simulink model "ClosedLoopSys"  (Simulink 8.4)
settings: Solver=ode1  StartTime=0.00  StopTime=60.00  FixedStep=T  RelTol=1e-5
values from neighbouring files (symbols this model uses):
  DAC_lim_l = 0    [heli.m]
  DAC_lim_u = 10    [heli.m]
  e_lim_l = -50*pi/180    (= -0.872664625997)    [heli.m]
  T = 0.015    [heli.m]
undefined symbols (not defined in the file or in its folder): Cr, kdfilt, Kdt, Kidt, U_e
settings Model: Creator=bjones  LastModifiedBy=bjones
settings DataIOCC: LimitDataPoints=off
settings OptimizationCC: BlockReduction=off  BooleanDataType=off
settings DebuggingCC: SaveWithParameterizedLinksMsg=none  SignalResolutionControl=TryResolveAllWithWarning  SolverPrmCheckMsg=none  MultiTaskDSMMsg=warning  MultiTaskCondExecSysMsg=none  StrictBusMsg=None
settings HardwareCC: TargetUnknown=on
settings RTWCC: IncludeERTFirstTime=on

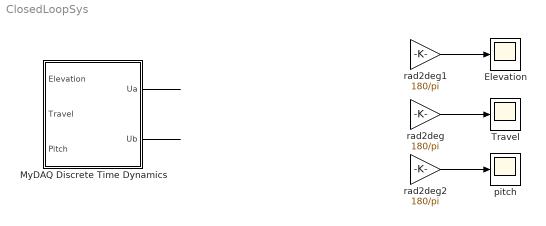
== system ClosedLoopSys ==
  Elevation : Scope
      settings: TimeRange=60  YMin=-50  YMax=30  SaveName=elev
  MyDAQ Discrete Time Dynamics : Subsystem
  Travel : Scope
      settings: TimeRange=60  YMin=-150  YMax=300  SaveName=trav
  pitch : Scope
      settings: TimeRange=60  YMin=-25  YMax=20  SaveName=pitch
  rad2deg : Gain  Gain=180/pi  SaturateOnIntegerOverflow=on  OutDataTypeStr=Inherit: Same as input  ParamDataTypeStr=Inherit: Same as input
  rad2deg1 : Gain  Gain=180/pi  SaturateOnIntegerOverflow=on  OutDataTypeStr=Inherit: Same as input  ParamDataTypeStr=Inherit: Same as input
  rad2deg2 : Gain  Gain=180/pi  SaturateOnIntegerOverflow=on  OutDataTypeStr=Inherit: Same as input  ParamDataTypeStr=Inherit: Same as input
  wires:
  rad2deg/1 -> Travel/1
  rad2deg1/1 -> Elevation/1
  ? -> MyDAQ Discrete Time Dynamics/2(Travel), rad2deg/1
  ? -> rad2deg1/1, MyDAQ Discrete Time Dynamics/1(Elevation)
  rad2deg2/1 -> pitch/1
  ? -> rad2deg2/1, MyDAQ Discrete Time Dynamics/3(Pitch)
  MyDAQ Discrete Time Dynamics/1(Ua) -> ?
  MyDAQ Discrete Time Dynamics/2(Ub) -> ?

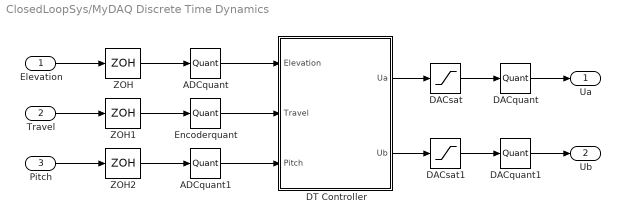
== system ClosedLoopSys/MyDAQ Discrete Time Dynamics ==
  Elevation : Inport
  Travel : Inport  Port=2
  Pitch : Inport  Port=3
  ADCquant : Quantizer  QuantizationInterval=ADC_Vres  SampleTime=T
  ADCquant1 : Quantizer  QuantizationInterval=ADC_Vres  SampleTime=T
  DACquant : Quantizer  QuantizationInterval=DAC_Vres  SampleTime=T
  DACquant1 : Quantizer  QuantizationInterval=DAC_Vres  SampleTime=T
  DACsat : Saturate  UpperLimit=DAC_lim_u  LowerLimit=DAC_lim_l  SampleTime=T
  DACsat1 : Saturate  UpperLimit=DAC_lim_u  LowerLimit=DAC_lim_l  SampleTime=T
  DT Controller : Subsystem
  Encoderquant : Quantizer  QuantizationInterval=Encoder_res  SampleTime=T
  ZOH : ZeroOrderHold  SampleTime=T
  ZOH1 : ZeroOrderHold  SampleTime=T
  ZOH2 : ZeroOrderHold  SampleTime=T
  Ua : Outport
  Ub : Outport  Port=2
  wires:
  Elevation/1 -> ZOH/1
  Travel/1 -> ZOH1/1
  DACquant/1 -> Ua/1
  DACquant1/1 -> Ub/1
  DT Controller/1(Ua) -> DACsat/1
  DACsat/1 -> DACquant/1
  DT Controller/2(Ub) -> DACsat1/1
  DACsat1/1 -> DACquant1/1
  ZOH1/1 -> Encoderquant/1
  ZOH/1 -> ADCquant/1
  Pitch/1 -> ZOH2/1
  ZOH2/1 -> ADCquant1/1
  ADCquant/1 -> DT Controller/1(Elevation)
  ADCquant1/1 -> DT Controller/3(Pitch)
  Encoderquant/1 -> DT Controller/2(Travel)

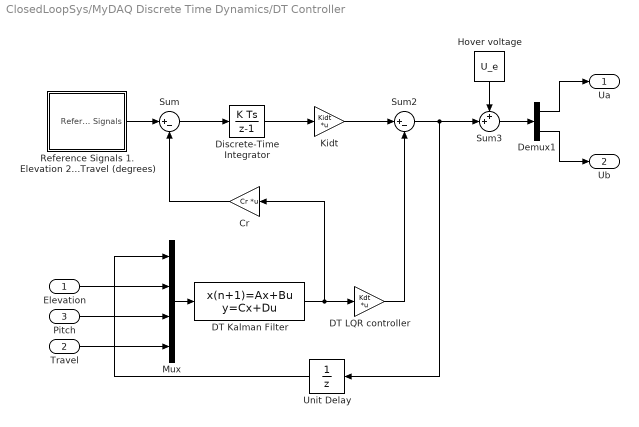
== system ClosedLoopSys/MyDAQ Discrete Time Dynamics/DT Controller ==
  Elevation : Inport
  Travel : Inport  Port=2
  Pitch : Inport  Port=3
  Cr : Gain  Gain=Cr  Multiplication=Matrix(K*u)
  DT Kalman Filter : DiscreteStateSpace  A=kdfilt.a  B=kdfilt.b  C=kdfilt.c(size(C,1)+1:end,:)  D=kdfilt.d(size(C,1)+1:end,:)  X0=[e_lim_l; 0; 0; 0; 0; 0]  SampleTime=T
  DT LQR controller : Gain  Gain=Kdt  Multiplication=Matrix(K*u)
  Demux1 : Demux  Outputs=2
  Discrete-Time Integrator : DiscreteIntegrator  SampleTime=T
  Hover voltage : Constant  Value=U_e  SampleTime=T
  Kidt : Gain  Gain=Kidt  Multiplication=Matrix(K*u)
  Mux : Mux
  Reference Signals 1. Elevation 2. Travel (degrees) : Subsystem
  Sum : Sum  Inputs=|+-  SampleTime=T
  Sum2 : Sum  Inputs=|+-  SampleTime=T
  Sum3 : Sum  Inputs=++|  SampleTime=T
  Unit Delay : UnitDelay  SampleTime=T
  Ua : Outport
  Ub : Outport  Port=2
  wires:
  Kidt/1 -> Sum2/1
  DT LQR controller/1 -> Sum2/2
  Hover voltage/1 -> Sum3/1
  Sum3/1 -> Demux1/1
  Demux1/1 -> Ua/1
  Demux1/2 -> Ub/1
  Sum2/1 -> Sum3/2, Unit Delay/1
  Discrete-Time Integrator/1 -> Kidt/1
  DT Kalman Filter/1 -> DT LQR controller/1, Cr/1
  Cr/1 -> Sum/2
  Mux/1 -> DT Kalman Filter/1
  Unit Delay/1 -> Mux/1
  Travel/1 -> Mux/4
  Pitch/1 -> Mux/3
  Elevation/1 -> Mux/2
  Reference Signals 1. Elevation 2. Travel (degrees)/1(Reference Signals) -> Sum/1
  Sum/1 -> Discrete-Time Integrator/1

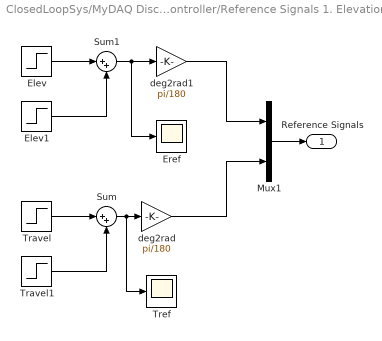
== system ClosedLoopSys/MyDAQ Discrete Time Dynamics/DT Controller/Reference Signals 1. Elevation 2. Travel (degrees) ==
  Elev : Step  Time=0  After=0  SampleTime=T
  Elev1 : Step  Time=30  After=10  SampleTime=T
  Eref : Scope
      settings: TimeRange=60  YMin=0  YMax=20  SaveName=eref
  Mux1 : Mux  Inputs=2
  Sum : Sum  Inputs=|++  SaturateOnIntegerOverflow=on  InputSameDT=on  OutDataTypeStr=Inherit: Same as first input
  Sum1 : Sum  Inputs=|++  SampleTime=T  SaturateOnIntegerOverflow=on  InputSameDT=on  OutDataTypeStr=Inherit: Same as first input
  Travel : Step  Time=10  After=180  SampleTime=T
  Travel1 : Step  Time=40  After=-180  SampleTime=T
  Tref : Scope
      settings: TimeRange=60  YMin=0  YMax=140  SaveName=tref
  deg2rad : Gain  Gain=pi/180  SaturateOnIntegerOverflow=on  OutDataTypeStr=Inherit: Same as input  ParamDataTypeStr=Inherit: Same as input
  deg2rad1 : Gain  Gain=pi/180  SaturateOnIntegerOverflow=on  OutDataTypeStr=Inherit: Same as input  ParamDataTypeStr=Inherit: Same as input
  Reference Signals : Outport
  wires:
  Travel/1 -> Sum/1
  Travel1/1 -> Sum/2
  Elev/1 -> Sum1/1
  Sum/1 -> deg2rad/1, Tref/1
  deg2rad/1 -> Mux1/2
  deg2rad1/1 -> Mux1/1
  Sum1/1 -> deg2rad1/1, Eref/1
  Elev1/1 -> Sum1/2
  Mux1/1 -> Reference Signals/1
